simulink model "TestingFile1"  (R2022b)
settings: Solver=VariableStepAuto  StartTime=0.0  StopTime=24  FixedStep=5e-9  MaxStep=0.01  RelTol=1e-3  AbsTol=1e-6
undefined symbols (not defined in the file): Acid, Lead
libraries: spsSeriesRLCBranchLib x24, spsCurrentMeasurementLib x19, spsIdealSwitchLib x10, spsMosfetLib x6, spsPWMGeneratorDCDCLib x5, spsDiodeLib x4, spsBatteryLib x2, slpidlib x2, spsIGBTLib x2, spsPVArrayLib x2, spsVoltageMeasurementLib x2, spspowerguiLib x1
(part 2 of 2)

== matlab function TestingFile1/MATLAB Function9 ==
  data: batt_status input; Vb_ref output; SOC input; Ib_ref output
function [Vb_ref, Ib_ref] = battery_reference_selector(batt_status, SOC)
% =========================================================================
%   FUNCTION 5: BATTERY REFERENCE SELECTOR  v3.0
%   Translates batt_status command → PI controller reference setpoints
% =========================================================================
%
% SYSTEM: 12V, 50Ah Lead-Acid Battery | Max current = 5A both directions
%
% WHAT IT DOES:
%   microgrid_optimization (FUNC4) makes the high-level decision:
%     +1 = "Charge the battery now"
%     -1 = "Discharge the battery now"
%      0 = "Leave the battery alone"
%
%   THIS function translates that command into exact voltage and current
%   references that your existing PI(z) controller can track.
%
%   The PI(z) controller then adjusts the duty cycle of the
%   bidirectional Buck/Boost converter to hit those targets.
%
% =========================================================================
% CHARGING PROFILE — 3-Stage CC/CV for Lead-Acid:
%
%   Stage 1 — BULK (SOC < 70%):
%     Vb_ref = 14.4V  →  drives max current into battery (PI clips at 5A)
%     Ib_ref = +5.0A  →  constant current, fastest safe charge rate
%     This is the stage triggered by the "battery as critical load" rule
%
%   Stage 2 — ABSORPTION (70% ≤ SOC < 90%):
%     Vb_ref = 13.8V  →  slightly lower, current starts tapering
%     Ib_ref = +3.0A  →  gentler charge as battery fills up
%
%   Stage 3 — FLOAT (SOC ≥ 90%):
%     Vb_ref = 13.2V  →  maintenance voltage only
%     Ib_ref = +1.0A  →  trickle to compensate self-discharge
%     (In practice batt_status=+1 is blocked at SOC≥90% by FUNC4,
%      this stage is a safety fallback only)
%
% DISCHARGING:
%   Vb_ref = 12.0V  →  hold bus at nominal 12V
%   Ib_ref = -5.0A  →  draw exactly 5A from battery (negative = out of battery)
%   PI(z) ensures current does not exceed 5A in discharge direction
%   This enforces: 50Ah ÷ 5A = 10 hours of backup
%
% IDLE (Float):
%   Vb_ref = 12.6V  →  typical lead-acid open-circuit voltage at ~50% SOC
%   Ib_ref =  0.0A  →  PI controller drives current to zero
%
% =========================================================================
% INPUTS:
%   batt_status — from FUNC4 output (+1 / -1 / 0)
%   SOC         — battery state of charge (%)
%
% OUTPUTS:
%   Vb_ref  — Voltage reference for voltage PI loop (Volts)
%             WIRING: Replace the Constant "12" block that currently feeds
%                     the (+) port of your voltage error Sum block
%   Ib_ref  — Current reference for current PI loop (Amps)
%             WIRING: Replace fixed Ib_ref constant at current Sum (+) port
%             Positive = charging into battery
%             Negative = discharging out of battery
% =========================================================================

    % Lead-Acid 12V voltage setpoints
    V_BULK       = 14.4;   % Bulk charge voltage (CC phase)
    V_ABSORB     = 13.8;   % Absorption voltage  (CV phase, tapering)
    V_FLOAT      = 13.2;   % Float voltage       (maintenance trickle)
    V_NOMINAL    = 12.0;   % Nominal discharge voltage
    V_IDLE       = 12.6;   % Open-circuit rest voltage (~50% SOC)

    % Current setpoints — 5A is the hard cap for 10-hr backup
    I_BULK       = +5.0;   % Amps — max charge rate (bulk stage)
    I_ABSORB     = +3.0;   % Amps — reduced charge rate (absorption stage)
    I_TRICKLE    = +1.0;   % Amps — maintenance trickle (float stage)
    I_DISCHARGE  = -5.0;   % Amps — max discharge (negative = out of battery)
    I_ZERO       =  0.0;   % Amps — idle, no current

    % SOC stage boundaries (must match FUNC4 constants)
    SOC_BULK_MAX    = 70;  % Bulk stage: SOC < 70%
    SOC_ABSORB_MAX  = 90;  % Absorption: 70% ≤ SOC < 90%
                            % Float:      SOC ≥ 90%

    % Default outputs (idle/safe)
    Vb_ref = V_IDLE;
    Ib_ref = I_ZERO;

    % ---------------------------------------------------------------
    if batt_status == 1
    % CHARGE MODE
    % ---------------------------------------------------------------
        if SOC < SOC_BULK_MAX
            % Stage 1 — BULK: Battery is low, charge at full 5A
            % This covers the "battery as critical load" scenario in FUNC4
            Vb_ref = V_BULK;
            Ib_ref = I_BULK;        % +5A → 60W → 10-hr backup guaranteed

        elseif SOC < SOC_ABSORB_MAX
            % Stage 2 — ABSORPTION: Battery getting full, taper down
            Vb_ref = V_ABSORB;
            Ib_ref = I_ABSORB;      % +3A → prevents gassing in lead-acid

        else
            % Stage 3 — FLOAT: Battery full, just maintain
            Vb_ref = V_FLOAT;
            Ib_ref = I_TRICKLE;     % +1A → trickle only
        end

    % ---------------------------------------------------------------
    elseif batt_status == -1
    % DISCHARGE MODE
    % ---------------------------------------------------------------
        % Hold bus at 12V nominal, draw max 5A from battery
        % Negative Ib_ref = current flowing OUT of battery
        Vb_ref = V_NOMINAL;
        Ib_ref = I_DISCHARGE;       % -5A → 60W → 10-hr backup

    % ---------------------------------------------------------------
    else
    % IDLE MODE (batt_status == 0)
    % ---------------------------------------------------------------
        % Hold battery at open-circuit rest voltage
        % PI controller drives current to zero → battery truly rests
        Vb_ref = V_IDLE;
        Ib_ref = I_ZERO;
    end

end

== matlab function TestingFile1/MATLAB Function10 ==
  data: batt_status input; Vb_ref output; SOC input; Ib_ref output
function [Vb_ref, Ib_ref] = battery_reference_selector(batt_status, SOC)
% =========================================================================
%   FUNCTION 5: BATTERY REFERENCE SELECTOR  v3.0
%   Translates batt_status command → PI controller reference setpoints
% =========================================================================
%
% SYSTEM: 12V, 50Ah Lead-Acid Battery | Max current = 5A both directions
%
% WHAT IT DOES:
%   microgrid_optimization (FUNC4) makes the high-level decision:
%     +1 = "Charge the battery now"
%     -1 = "Discharge the battery now"
%      0 = "Leave the battery alone"
%
%   THIS function translates that command into exact voltage and current
%   references that your existing PI(z) controller can track.
%
%   The PI(z) controller then adjusts the duty cycle of the
%   bidirectional Buck/Boost converter to hit those targets.
%
% =========================================================================
% CHARGING PROFILE — 3-Stage CC/CV for Lead-Acid:
%
%   Stage 1 — BULK (SOC < 70%):
%     Vb_ref = 14.4V  →  drives max current into battery (PI clips at 5A)
%     Ib_ref = +5.0A  →  constant current, fastest safe charge rate
%     This is the stage triggered by the "battery as critical load" rule
%
%   Stage 2 — ABSORPTION (70% ≤ SOC < 90%):
%     Vb_ref = 13.8V  →  slightly lower, current starts tapering
%     Ib_ref = +3.0A  →  gentler charge as battery fills up
%
%   Stage 3 — FLOAT (SOC ≥ 90%):
%     Vb_ref = 13.2V  →  maintenance voltage only
%     Ib_ref = +1.0A  →  trickle to compensate self-discharge
%     (In practice batt_status=+1 is blocked at SOC≥90% by FUNC4,
%      this stage is a safety fallback only)
%
% DISCHARGING:
%   Vb_ref = 12.0V  →  hold bus at nominal 12V
%   Ib_ref = -5.0A  →  draw exactly 5A from battery (negative = out of battery)
%   PI(z) ensures current does not exceed 5A in discharge direction
%   This enforces: 50Ah ÷ 5A = 10 hours of backup
%
% IDLE (Float):
%   Vb_ref = 12.6V  →  typical lead-acid open-circuit voltage at ~50% SOC
%   Ib_ref =  0.0A  →  PI controller drives current to zero
%
% =========================================================================
% INPUTS:
%   batt_status — from FUNC4 output (+1 / -1 / 0)
%   SOC         — battery state of charge (%)
%
% OUTPUTS:
%   Vb_ref  — Voltage reference for voltage PI loop (Volts)
%             WIRING: Replace the Constant "12" block that currently feeds
%                     the (+) port of your voltage error Sum block
%   Ib_ref  — Current reference for current PI loop (Amps)
%             WIRING: Replace fixed Ib_ref constant at current Sum (+) port
%             Positive = charging into battery
%             Negative = discharging out of battery
% =========================================================================

    % Lead-Acid 12V voltage setpoints
    V_BULK       = 14.4;   % Bulk charge voltage (CC phase)
    V_ABSORB     = 13.8;   % Absorption voltage  (CV phase, tapering)
    V_FLOAT      = 13.2;   % Float voltage       (maintenance trickle)
    V_NOMINAL    = 12.0;   % Nominal discharge voltage
    V_IDLE       = 12.6;   % Open-circuit rest voltage (~50% SOC)

    % Current setpoints — 5A is the hard cap for 10-hr backup
    I_BULK       = +5.0;   % Amps — max charge rate (bulk stage)
    I_ABSORB     = +3.0;   % Amps — reduced charge rate (absorption stage)
    I_TRICKLE    = +1.0;   % Amps — maintenance trickle (float stage)
    I_DISCHARGE  = -5.0;   % Amps — max discharge (negative = out of battery)
    I_ZERO       =  0.0;   % Amps — idle, no current

    % SOC stage boundaries (must match FUNC4 constants)
    SOC_BULK_MAX    = 70;  % Bulk stage: SOC < 70%
    SOC_ABSORB_MAX  = 90;  % Absorption: 70% ≤ SOC < 90%
                            % Float:      SOC ≥ 90%

    % Default outputs (idle/safe)
    Vb_ref = V_IDLE;
    Ib_ref = I_ZERO;

    % ---------------------------------------------------------------
    if batt_status == 1
    % CHARGE MODE
    % ---------------------------------------------------------------
        if SOC < SOC_BULK_MAX
            % Stage 1 — BULK: Battery is low, charge at full 5A
            % This covers the "battery as critical load" scenario in FUNC4
            Vb_ref = V_BULK;
            Ib_ref = I_BULK;        % +5A → 60W → 10-hr backup guaranteed

        elseif SOC < SOC_ABSORB_MAX
            % Stage 2 — ABSORPTION: Battery getting full, taper down
            Vb_ref = V_ABSORB;
            Ib_ref = I_ABSORB;      % +3A → prevents gassing in lead-acid

        else
            % Stage 3 — FLOAT: Battery full, just maintain
            Vb_ref = V_FLOAT;
            Ib_ref = I_TRICKLE;     % +1A → trickle only
        end

    % ---------------------------------------------------------------
    elseif batt_status == -1
    % DISCHARGE MODE
    % ---------------------------------------------------------------
        % Hold bus at 12V nominal, draw max 5A from battery
        % Negative Ib_ref = current flowing OUT of battery
        Vb_ref = V_NOMINAL;
        Ib_ref = I_DISCHARGE;       % -5A → 60W → 10-hr backup

    % ---------------------------------------------------------------
    else
    % IDLE MODE (batt_status == 0)
    % ---------------------------------------------------------------
        % Hold battery at open-circuit rest voltage
        % PI controller drives current to zero → battery truly rests
        Vb_ref = V_IDLE;
        Ib_ref = I_ZERO;
    end

end

== matlab function TestingFile1/MATLAB Function11 ==
  settings: updateMethod=DISCRETE
  data: P_pv input; SOC input; r1 output; r2 output; r3 output; r4 output; r5 output; batt_status output; sw1 input; sw2 input; sw3 input; sw4 input; sw5 input; Hour input
function [r1, r2, r3, r4, r5, batt_status] = nanogrid_opt_ilp( ...
    P_pv, SOC, sw1, sw2, sw3, sw4, sw5, Hour)

% =========================================================================
% ILP-INSPIRED NANOGRID OPTIMIZER (Simulink Compatible)
% =========================================================================

%% CONSTANTS
Load_W = [60, 20, 100, 60, 20];   % [Fan1 Bulb1 Pump Fan2 Bulb2]
Weights = [1000, 1000, 10, 10, 10]; % Priority weights

SOC_HIGH = 90;
SOC_LOW  = 40;
SOC_FLOOR = 5;

BATT_W = 60;

NIGHT_START = 20;
NIGHT_END   = 6;

SW = [sw1, sw2, sw3, sw4, sw5];
is_Night = (Hour >= NIGHT_START) || (Hour < NIGHT_END);

%% SEARCH SPACE
best_J = 1e9;
best_relays = [0 0 0 0 0];
best_batt = 0;

% 32 combinations (5 loads)
for i = 0:31
    
    % Candidate relay vector
    x = zeros(1,5);
    for b = 1:5
        x(b) = bitget(i, b);
    end
    
    %% ==============================
    % HARD CONSTRAINTS
    % ==============================
    valid = true;
    
    % Cannot turn ON load if user switch OFF
    for k = 1:5
        if x(k) == 1 && SW(k) == 0
            valid = false;
        end
    end
    
    % DAY: NC loads forbidden
    if ~is_Night
        if x(3) || x(4) || x(5)
            valid = false;
        end
    end
    
    % NIGHT: Pump & Fan2 forbidden
    if is_Night
        if x(3) || x(4)
            valid = false;
        end
    end
    
    if ~valid
        continue;
    end
    
    %% ==============================
    % POWER CALCULATION
    % ==============================
    P_load = sum(x .* Load_W);
    
    % Battery requirement
    P_batt_needed = P_load - P_pv;
    
    batt = 0;
    
    % Battery feasibility
    if P_batt_needed > 0
        % Discharging
        if SOC <= SOC_LOW
            valid = false;
        elseif P_batt_needed > BATT_W
            valid = false;
        else
            batt = -1;
        end
        
    else
        % Charging
        if SOC >= SOC_HIGH
            batt = 0;
        else
            batt = 1;
        end
    end
    
    if ~valid
        continue;
    end
    
    %% ==============================
    % COST FUNCTION (THE CORE)
    % ==============================
    
    % 1. Load shedding penalty
    shed_cost = 0;
    for k = 1:5
        shed_cost = shed_cost + Weights(k) * (SW(k) - x(k));
    end
    
    % 2. Battery usage penalty
    batt_cost = 0.2 * abs(P_batt_needed);
    
    % 3. SOC protection penalty
    soc_penalty = 0;
    if SOC < 50 && batt == -1
        soc_penalty = 500;
    end
    
    % 4. Night preference (limit loads)
    night_penalty = 0;
    if is_Night && sum(x) > 1
        night_penalty = 200;
    end
    
    % FINAL COST
    J = shed_cost + batt_cost + soc_penalty + night_penalty;
    
    %% ==============================
    % MINIMIZATION
    % ==============================
    if J < best_J
        best_J = J;
        best_relays = x;
        best_batt = batt;
    end
end

%% OUTPUTS
r1 = best_relays(1);
r2 = best_relays(2);
r3 = best_relays(3);
r4 = best_relays(4);
r5 = best_relays(5);
batt_status = best_batt;

%% SAFETY OVERRIDES
if SOC <= SOC_FLOOR
    r1=0; r2=0; r3=0; r4=0; r5=0;
    batt_status = 0;
end

if SOC >= SOC_HIGH && batt_status == 1
    batt_status = 0;
end

if SOC <= SOC_LOW && batt_status == -1
    batt_status = 0;
end

end

== matlab function TestingFile1/MATLAB Function1 ==
  data: I_flow input; G1_to_G2 output; G2_to_G1 output
function [G1_to_G2, G2_to_G1] = checkPowerDirection(I_flow)

% Small deadband to avoid noise-triggered switching
I_threshold = 0.01;   % 10 mA tolerance (adjust as needed)

% Default outputs
G1_to_G2 = 0;
G2_to_G1 = 0;

if I_flow > I_threshold
    G1_to_G2 = 1;

elseif I_flow < -I_threshold
    G2_to_G1 = 1;

else
    % Within deadband → no transfer
    G1_to_G2 = 0;
    G2_to_G1 = 0;
end

end

== matlab function TestingFile1/MATLAB Function ==
  data: P_new input; Y output; P_old input; Delay input; Yin input; Stage_in input; Stage_out output; Pold_out output
function [Y,Stage_out,Pold_out]=MPPT(P_new,P_old,Delay,Yin,Stage_in) 

c=0.05;

Pold_out=P_old;

Y=Yin;

Stage_out= Stage_in;

if Delay == 0

    if Stage_in==0

                    if  P_new>P_old

                    Y=Yin+c;

                    Pold_out=P_new;

                    elseif P_new<P_old

                    Y=Yin-c;

                    Stage_out=1;

                    Pold_out=P_new;

                    end

                    Pold_out=P_new;

    end

   if Stage_in==1

                    if P_new>P_old

                    Y=Yin-c;

                     Pold_out=P_new;

                    elseif P_new<P_old

                    Y=Yin+c;

                    Stage_out=0;

                    Pold_out=P_new;

                    end

                    Pold_out=P_new;

   end           

end

== matlab function TestingFile1/MATLAB Function2 ==
  settings: updateMethod=DISCRETE
  data: duty output; P_transfer output; V1 input; V2 input; SOC1 input; SOC2 input; Pload1 input; Pload2 input; PPV1 input; PPV2 input; Hour input
function [duty, P_transfer] = duty_controller_opt( ...
    V1, V2, SOC1, SOC2, Pload1, Pload2, PPV1, PPV2, Hour)

% =========================================================================
% OPTIMIZATION-BASED INTER-GRID CONTROLLER (Simulink Compatible)
% Inspired by ILP but implemented as discrete search (fast & safe)
% =========================================================================

%% Constants
Duty_base        = 0.5;
Duty_max_offset  = 0.25;
Converter_Rating = 300;
Power_margin     = 60;
V_diff_thresh    = 0.5;

SOC_NO_EXPORT = 50;
SOC_NO_IMPORT = 70;

NIGHT_START = 20;
NIGHT_END   = 6;

%% Default
duty = Duty_base;
P_transfer = 0;

%% Night condition (same as before)
if (Hour >= NIGHT_START) || (Hour < NIGHT_END)
    return;
end

%% Net power
Net1 = PPV1 - Pload1;
Net2 = PPV2 - Pload2;

%% Decision variables:
% x = -1 → Grid2 → Grid1
% x =  0 → No transfer
% x = +1 → Grid1 → Grid2

best_cost = 1e9;
best_x = 0;

for x = [-1, 0, 1]

    cost = 0;
    valid = true;

    if x == 1
        % Grid1 → Grid2
        
        if ~(Net1 > Power_margin)
            valid = false;
        end
        if ~(SOC1 >= SOC_NO_EXPORT)
            valid = false;
        end
        if ~(SOC2 <= SOC_NO_IMPORT)
            valid = false;
        end
        if ~(V1 > V2 + V_diff_thresh)
            valid = false;
        end
        
        % Cost: prefer using surplus
        cost = -Net1;

    elseif x == -1
        % Grid2 → Grid1
        
        if ~(Net2 > Power_margin)
            valid = false;
        end
        if ~(SOC2 >= SOC_NO_EXPORT)
            valid = false;
        end
        if ~(SOC1 <= SOC_NO_IMPORT)
            valid = false;
        end
        if ~(V2 > V1 + V_diff_thresh)
            valid = false;
        end
        
        cost = -Net2;

    else
        % No transfer
        cost = 10; % small penalty to encourage sharing
    end

    if valid && cost < best_cost
        best_cost = cost;
        best_x = x;
    end
end

%% Apply best decision
if best_x == 1
    duty_offset = Duty_max_offset * min(1.0, Net1 / Converter_Rating);
    duty = Duty_base + duty_offset;
    P_transfer = duty_offset * Converter_Rating / Duty_max_offset;

elseif best_x == -1
    duty_offset = Duty_max_offset * min(1.0, Net2 / Converter_Rating);
    duty = Duty_base - duty_offset;
    P_transfer = -duty_offset * Converter_Rating / Duty_max_offset;

else
    duty = Duty_base;
    P_transfer = 0;
end

%% Clamp
duty = max(0.05, min(0.95, duty));

end

== matlab function TestingFile1/MATLAB Function3 ==
  data: P_new input; Y output; P_old input; Delay input; Yin input; Stage_in input; Stage_out output; Pold_out output
function [Y,Stage_out,Pold_out]=MPPT(P_new,P_old,Delay,Yin,Stage_in) 

c=0.05;

Pold_out=P_old;

Y=Yin;

Stage_out= Stage_in;

if Delay == 0

    if Stage_in==0

                    if  P_new>P_old

                    Y=Yin+c;

                    Pold_out=P_new;

                    elseif P_new<P_old

                    Y=Yin-c;

                    Stage_out=1;

                    Pold_out=P_new;

                    end

                    Pold_out=P_new;

    end

   if Stage_in==1

                    if P_new>P_old

                    Y=Yin-c;

                     Pold_out=P_new;

                    elseif P_new<P_old

                    Y=Yin+c;

                    Stage_out=0;

                    Pold_out=P_new;

                    end

                    Pold_out=P_new;

   end           

end

== matlab function TestingFile1/MATLAB Function4 ==
  settings: updateMethod=DISCRETE
  data: t input; day_type output; G_meas input
function day_type = forecast_selector(t, G_meas)
% day_type:
% 1 = Summer
% 2 = Winter
% 3 = Cloudy

% Persistent variables (memory)
persistent G_peak G_prev
if isempty(G_peak)
    G_peak = 0;
    G_prev = G_meas;
end

% Track maximum irradiance observed
G_peak = max(G_peak, G_meas);

% Detect cloud-induced fluctuation
G_change = abs(G_meas - G_prev);
G_prev = G_meas;

% --- Decision logic ---

% Cloudy day: frequent large fluctuations
if G_change > 150
    day_type = 3;   % Cloudy
    return;
end

% Seasonal classification by peak irradiance
if G_peak >= 850
    day_type = 1;   % Summer
elseif G_peak >= 500
    day_type = 2;   % Winter
else
    day_type = 3;   % Cloudy
end

== matlab function TestingFile1/MATLAB Function5 ==
  data: t input; G output; day_type input
function G = irradiance_generator(t, day_type)
% Generates irradiance based on selected day type

T = (0:23);

G_summer = [ ...
    0 0 0 0 0 50 150 300 500 700 850 950 ...
    1000 980 900 750 600 400 200 80 0 0 0 0 ];

G_winter = [ ...
    0 0 0 0 0 0 0 50 150 300 450 600 ...
    700 650 500 350 200 80 0 0 0 0 0 0 ];

G_cloudy = [ ...
    0 0 0 0 0 0 60 120 250 400 300 450 ...
    500 350 420 280 180 90 30 0 0 0 0 0 ];

% Select profile
if day_type == 1
    G_table = G_summer;
elseif day_type == 2
    G_table = G_winter;
else
    G_table = G_cloudy;
end

% Time saturation
t = min(max(t,0), T(end));

% Interpolated irradiance
G = interp1(T, G_table, t);

== matlab function TestingFile1/MATLAB Function6 ==
  settings: updateMethod=DISCRETE
  data: t input; day_type output; G_meas input
function day_type = forecast_selector(t, G_meas)
% day_type:
% 1 = Summer
% 2 = Winter
% 3 = Cloudy

% Persistent variables (memory)
persistent G_peak G_prev
if isempty(G_peak)
    G_peak = 0;
    G_prev = G_meas;
end

% Track maximum irradiance observed
G_peak = max(G_peak, G_meas);

% Detect cloud-induced fluctuation
G_change = abs(G_meas - G_prev);
G_prev = G_meas;

% --- Decision logic ---

% Cloudy day: frequent large fluctuations
if G_change > 150
    day_type = 3;   % Cloudy
    return;
end

% Seasonal classification by peak irradiance
if G_peak >= 850
    day_type = 1;   % Summer
elseif G_peak >= 500
    day_type = 2;   % Winter
else
    day_type = 3;   % Cloudy
end
